simulink model "aula_08_lab"  (R2024a)
settings: Solver=VariableStepAuto  StartTime=0.0  StopTime=tsim  MaxStep=1e-1  RelTol=1e-3
values from neighbouring files (symbols this model uses):
  ae0 = 0.6    [Lab11.m]    (also in Lab11_pronto.m; Lab_7.m; aula08.m; aula08_lab.m)
  as0 = 0.5    [Lab11.m]    (also in Lab11_pronto.m; Lab_7.m; aula08.m; aula08_lab.m)
  gamma = 1/8    (= 0.125)    [Lab11.m]    (also in Lab11_pronto.m; aula08.m; aula08_lab.m; lab09.m)
  H0 = ((ke*ae0)/(ks*as0*sqrt(2*g)))^2    [Lab11.m]    (also in Lab11_pronto.m = ((ke*ae0)/(ks*as0*sqrt(2*gg)))^2; Lab_7.m; aula08.m; aula08_lab.m)
  H_ref = H0 + 0.10    [Lab11_pronto.m]    (also in Lab_7.m; aula08.m; aula08_lab.m)
  Kc = 0.2587    [Lab11.m]    (also in Lab11_pronto.m; aula08.m = 3; aula08_lab.m = 1; lab09.m = M(idx).Kc)
  Td = 20.66    [Lab11.m]    (also in Lab11_pronto.m; aula08.m = 0; aula08_lab.m = 0; lab09.m = M(idx).Td)
  Ti = 53.90    (= 53.9)    [Lab11.m]    (also in Lab11_pronto.m; aula08.m = 1.2; aula08_lab.m = 20; lab09.m = M(idx).Ti)
  tsim = 2500    [Lab11.m]    (also in Lab11_pronto.m; Lab_7.m = 500; aula08.m = 500; aula08_lab.m = 500)
libraries: cstblocks x3
settings Model: Creator=Prof. Daniel Cruz  LastModifiedBy=Prof. Daniel Cruz
settings SolverCC: AlgebraicLoopSolver=TrustRegion
settings DebuggingCC: UnconnectedInputMsg=warning  UnconnectedOutputMsg=warning  UnconnectedLineMsg=warning
settings ModelReferenceCC: EnableRefExpFcnMdlSchedulingChecks=on
settings RTWCC: GPUComputeCapability=3.5

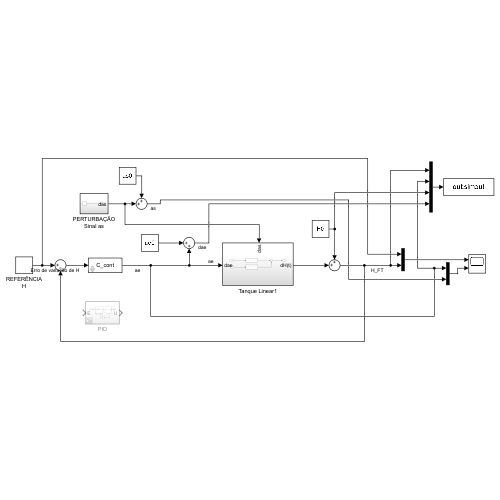
[thumbnail: Simulink's stored preview of the top-level diagram]
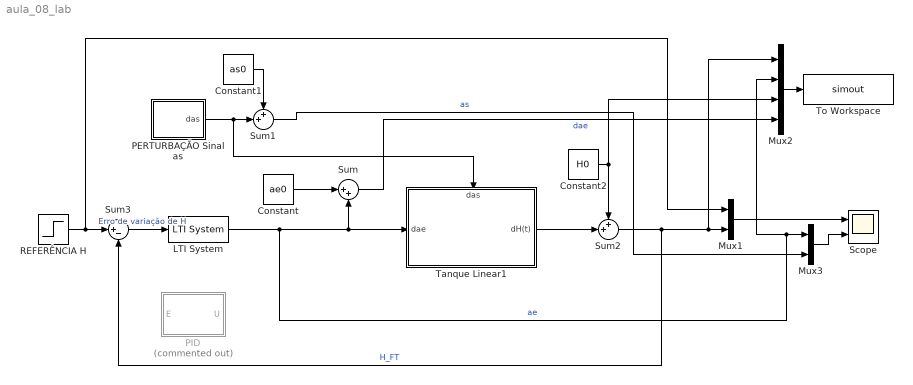
== system aula_08_lab ==
  Constant : Constant  Value=ae0
  Constant1 : Constant  Value=as0
  Constant2 : Constant  Value=H0
  LTI System : cstblocks/LTI System  sys=C_cont  IC=[]  PadeOrder=0
  Mux1 : Mux  Inputs=2
  Mux2 : Mux
  Mux3 : Mux  Inputs=2
  PERTURBAÇÃO Sinal as : Subsystem
  PID : Subsystem  Commented=on
  REFERÊNCIA H : Step  Time=0  Before=H0  After=H_ref  SampleTime=0
  Scope : Scope  NumInputPorts=2
  Sum : Sum  Inputs=|++
  Sum1 : Sum  Inputs=++|
  Sum2 : Sum  Inputs=++|
  Sum3 : Sum  Inputs=|+-
  Tanque Linear1 : Subsystem
      settings: PortSchema="{\"entries\":[{\"content\":{\"sides\":[{\"content\":{\"connectorIds\":[\"In1\"]},\"type\":\"ConnectorPlacement.EquallySpacedRectSide\",\"uuid\":\"f67b16a6-d13c-4ce1-92bf-a3b7b78f55b2\"},{\"content\":{\"connectorIds\":[\"Out1\"],\"side\":\"RIGHT\"},\"type\":\"ConnectorPlacement.EquallySpacedRectSide\",\"uuid\":\"6dfa0371-c497-4466-b77b-e5c5fe181385\"},{\"content\":{\"connectorIds\":[\"In2\"],\"side\":\"TOP\"},\"type\":\"ConnectorPlacement.EquallySpacedRectSide\",\"uuid\":\"6450f77e-1436-4798-86e5-b0a6495bdb9b\"}]},\"type\":\"ConnectorPlacement.EquallySpacedConnector\",\"uuid\":\"6402b57b-709e-4d3a-bcb1-330d3ba010a6\"}],\"packageUris\":[\"http://schema.mathworks.com/mf0/Connector/R2020b\"],\"version\":\"1.0\"}"
  To Workspace : ToWorkspace  VariableName=simout  SaveFormat=Timeseries  SampleTime=-1
  wires:
  Constant/1 -> Sum/1
  Constant1/1 -> Sum1/1
  PERTURBAÇÃO Sinal as/1(das) -> Tanque Linear1/2(das), Sum1/2
  Tanque Linear1/1(dH(t)) -> Sum2/2
  Constant2/1 -> Sum2/1, Mux2/3
  Sum2/1 -> Sum3/2, Mux2/1, Mux1/2  "H_FT"
  Mux1/1 -> Scope/1
  Sum1/1 -> Mux3/2  "as"
  REFERÊNCIA H/1 -> Mux1/1, Sum3/1
  Sum3/1 -> LTI System/1  "Erro de variação de H"
  LTI System/1 -> Tanque Linear1/1(dae), Sum/2, Mux3/1, Mux2/2  "ae"
  Mux2/1 -> To Workspace/1
  Mux3/1 -> Scope/2
  Sum/1 -> Mux2/4  "dae"

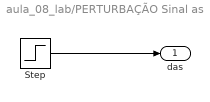
== system aula_08_lab/PERTURBAÇÃO Sinal as ==
  Step : Step  Time=(4/8)*tsim  After=0.1  SampleTime=0
  das : Outport
  wires:
  Step/1 -> das/1

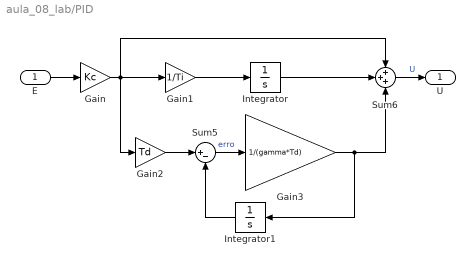
== system aula_08_lab/PID ==
  E : Inport
  Gain : Gain  Gain=Kc
  Gain1 : Gain  Gain=1/Ti
  Gain2 : Gain  Gain=Td
  Gain3 : Gain  Gain=1/(gamma*Td)
  Integrator : Integrator
  Integrator1 : Integrator
  Sum5 : Sum  Inputs=|+-
  Sum6 : Sum  Inputs=+++
  U : Outport
  wires:
  Gain2/1 -> Sum5/1
  Gain3/1 -> Integrator1/1, Sum6/3
  Gain/1 -> Gain1/1, Sum6/1, Gain2/1
  Integrator1/1 -> Sum5/2
  Integrator/1 -> Sum6/2
  Sum5/1 -> Gain3/1  "erro"
  Sum6/1 -> U/1  "U"
  Gain1/1 -> Integrator/1
  E/1 -> Gain/1

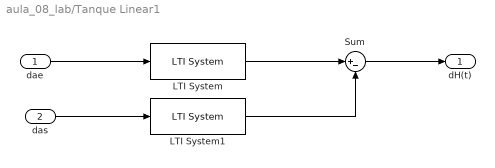
== system aula_08_lab/Tanque Linear1 ==
  dae : Inport
  das : Inport  Port=2
  LTI System : cstblocks/LTI System  sys=G  IC=[]  PadeOrder=0
  LTI System1 : cstblocks/LTI System  sys=Gas  IC=[]  PadeOrder=0
  Sum : Sum  Inputs=|+-
  dH(t) : Outport
  wires:
  dae/1 -> LTI System/1
  das/1 -> LTI System1/1
  LTI System/1 -> Sum/1
  LTI System1/1 -> Sum/2
  Sum/1 -> dH(t)/1
